simulink model "VoltageSourceConverterHVDCTrans"  (R2025b)
settings: Solver=FixedStepDiscrete  StartTime=0.0  StopTime=5  FixedStep=Ts  MaxStep=1e-4  RelTol=1e-3
PreLoadFcn:
  | VoltageSourceConverterHVDCTransParameters
values from neighbouring files (symbols this model uses):
  c = 0.207e-6    (= 2.07e-07)    [VoltageSourceConverterHVDCTransParameters.m]
  Cf = ((QRatedFilter/(VRated^2*(2*pi*FRated)))*(n^2-1)/(n^2))/Cbase    [VoltageSourceConverterHVDCTransParameters.m]
  FRated = 60    [VoltageSourceConverterHVDCTransParameters.m]
  Idcbase = Pbase/VdcRated    (= 1000)    [VoltageSourceConverterHVDCTransParameters.m]
  IL0 = opIdc.get("I").Value.value    [VoltageSourceConverterHVDCTransInitializeModel.m]
  l = 0.189e-3    (= 0.000189)    [VoltageSourceConverterHVDCTransParameters.m]
  Lbase = Zbase/wbase    [VoltageSourceConverterHVDCTransParameters.m]
  Lr = 0.15    [VoltageSourceConverterHVDCTransParameters.m]
  n = 25    [VoltageSourceConverterHVDCTransParameters.m]
  PRated = 300e6    (= 300000000)    [VoltageSourceConverterHVDCTransParameters.m]
  r = 0.0376    [VoltageSourceConverterHVDCTransParameters.m]
  Rc = r*Dis    (= 11.28)    [VoltageSourceConverterHVDCTransParameters.m]
  Rr = 0.002    [VoltageSourceConverterHVDCTransParameters.m]
  Rt = 0.002625    [VoltageSourceConverterHVDCTransParameters.m]
  Ts = 1/(fsw*100)    [VoltageSourceConverterHVDCTransInitializeModel.m]    (also in VoltageSourceConverterHVDCTransParameters.m = 6.66666666667e-05; VoltageSourceConverterHVDCTransVariantControl.m)
  Tsc = 10*Ts    (= 0.166666666667)    [VoltageSourceConverterHVDCTransInitializeModel.m]    (also in VoltageSourceConverterHVDCTransParameters.m = 6.66666666667e-05; VoltageSourceConverterHVDCTransVariantControl.m)
  Vdcr0 = 2*opReceivingEndVdcp.get("V").Value.value    [VoltageSourceConverterHVDCTransInitializeModel.m]
  VdcRated = 300e3    (= 300000)    [VoltageSourceConverterHVDCTransParameters.m]
  Vdcs0 = 2*opSendingEndVdcp.get("V").Value.value    [VoltageSourceConverterHVDCTransInitializeModel.m]
  VRated = 150e3    (= 150000)    [VoltageSourceConverterHVDCTransParameters.m]
  Xt = 0.19197    [VoltageSourceConverterHVDCTransParameters.m]
  Zbase = Vbase/Ibase    [VoltageSourceConverterHVDCTransParameters.m]
undefined symbols (not defined in the file or in its folder): DiscIntNeverNeededParam
libraries: nesl_utility x43, fl_lib x32, ee_lib x22, eeTransforms x16, eeGeneralControl x14, slpidlib x13, mcbeeMathTransformLib x8, eeSinusoidalMeasurement x2, eePwmGeneratorThreeLevel x2
(part 1 of 4)
CloseFcn:
  | try,close(h1_VoltageSourceConverterHVDCTrans),end
  | clear h1_VoltageSourceConverterHVDCTrans
  | 
  | clear
settings Model: Creator=The MathWorks, Inc.  LastModifiedBy=Elvin
settings DataIOCC: InspectSignalLogs=on  ReturnWorkspaceOutputs=off  SignalLoggingName=logsout_VoltageSourceConverterHVDCTrans
settings DebuggingCC: SubsystemReferenceDiagnosticForUnitTest=warning
settings RTWCC: GPUComputeCapability=3.5
settings SimscapeCC: SimscapeLogType=all  SimscapeLogName=simlog_VoltageSourceConverterHVDCTrans  SimscapeLogLimitData=off  SimscapeOperatingPoint=op

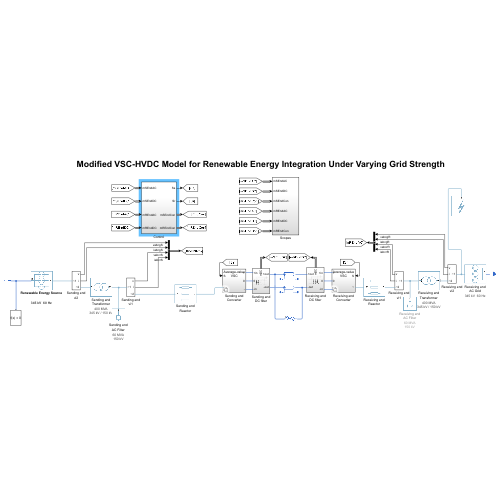
[thumbnail: Simulink's stored preview of the top-level diagram]
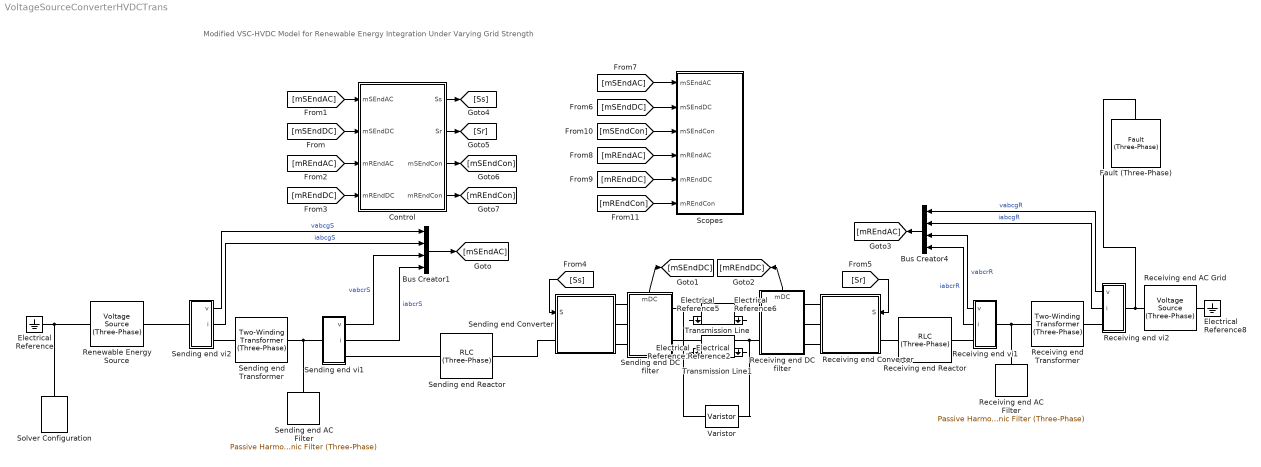
== system VoltageSourceConverterHVDCTrans ==
  note: Modified VSC-HVDC Model for Renewable Energy Integration Under Varying Grid Strength
  Bus Creator1 : BusCreator  Inputs=4
  Bus Creator4 : BusCreator  Inputs=4
  Control : Subsystem
  Electrical Reference{,1..2,5..6,8} (6 alike) : fl_lib/Electrical/Electrical Elements/Electrical Reference
  Fault (Three-Phase) : ee_lib/Utilities/Fault (Three-Phase)  fault_type_option=10  R_pn_fault=0.04 Ohm  R_ng_fault=1e-3 Ohm  exposemeasurement=ee.enum.exposemeasurement.hidden  enable_external_fault=ee.enum.external_fault.hidden  fault_threshold=0.5  fault_condition=1  fault_resettable=0  enable_temporal_fault=1  fault_start_time=2 s  fault_duration=140 ms  G_parasitic=1e-6 1/Ohm
      settings: InternalSimscapePortConfiguration="{\"Bottom\":[],\"Left\":[{\"id\":\"N\",\"label\":\"~\",\"type\":\"foundation.electrical.three_phase\"}],\"Right\":[],\"Top\":[]}"
  Receiving end AC Filter : ee_lib/Passive/Passive Harmonic Filter (Three-Phase)  QRated=QRatedFilter A*V  VRated=VRated V  FRated=FRated Hz  qfactor=15  type_option=ee.enum.filtertype.HPsecondorder  connection_option=ee.enum.filterconnection.Yg  ftuned=n*60 Hz  ftuned1=7 * 60 Hz  ftuned2=11 * 60 Hz  I_specify=off  I_priority=None  I=[0, 0, 0] A  I_nominal_specify=off  I_nominal_value=1  I_nominal_unit=A  V_specify=off  V_priority=None  V=[0, 0, 0] V  V_nominal_specify=off  V_nominal_value=1  V_nominal_unit=V
      settings: InternalSimscapePortConfiguration="{\"Bottom\":[],\"Left\":[{\"id\":\"N\",\"label\":\"~\",\"type\":\"foundation.electrical.three_phase\"}],\"Right\":[],\"Top\":[]}"
      settings: AttributesFormatString=|
      | 60 MVA
      | 150 kV
  Receiving end AC Grid : ee_lib/Sources/Voltage Source (Three-Phase)  vline_rms=VgridRated1 V  shift=0 deg  freq=FRated Hz  impedance_option=1  SShortCircuit=1500e6 A*V  XR=10  R=0.01 Ohm  L=3.97e-4 H  harmonic_option=0  harmonic_orders=[5, 7, 11, 13]  harmonic_ratios=[.1, .1, .1, .1]  G_parasitic=0 1/Ohm  I_specify=on  I_priority=None  I=[0, 0, 0] A  I_nominal_specify=on  I_nominal_value=1  I_nominal_unit=A
      settings: AttributesFormatString="345 kV  60 Hz"
  Receiving end Converter : Subsystem  Variant=on
  Receiving end DC filter : Subsystem
      settings: PortSchema="{\"entries\":[{\"content\":{\"sides\":[{\"content\":{\"connectorIds\":[\"LConn1\",\"LConn2\"]},\"type\":\"ConnectorPlacement.EquallySpacedRectSide\",\"uuid\":\"66d4cfbf-dcba-4749-bf5d-5811a775276e\"},{\"content\":{\"connectorIds\":[\"RConn1\",\"RConn2\",\"RConn3\"],\"side\":\"RIGHT\"},\"type\":\"ConnectorPlacement.EquallySpacedRectSide\",\"uuid\":\"35abdffa-cda0-46f2-9903-3f86a9532248\"},{\"content\":{\"connectorIds\":[\"Out1\"],\"side\":\"TOP\"},\"type\":\"ConnectorPlacement.EquallySpacedRectSide\",\"uuid\":\"3c5502e5-1b76-444d-b26b-a5789383a319\"}]},\"type\":\"ConnectorPlacement.EquallySpacedConnector\",\"uuid\":\"b78b2c4f-7eb3-43f3-aa61-891430661a3a\"}],\"packageUris\":[\"http://schema.mathworks.com/mf0/Connector/R2020b\"],\"version\":\"1.0\"}"
  Receiving end Reactor : ee_lib/Passive/RLC Assemblies/RLC (Three-Phase)  port_option=ee.enum.threePhasePort.composite  component_structure=ee.enum.rlc.structure.SeriesRL  R=Rr*Zbase Ohm  L=Lr*Lbase H  C=1e-6 F  R_parasitic=0 Ohm  G_parasitic=0 1/Ohm  IL_specify=off  IL_priority=High  IL=[0, 0, 0] A  IL_nominal_specify=on  IL_nominal_value=1  IL_nominal_unit=A  VC_specify=off  VC_priority=High  VC=[0, 0, 0] V  VC_nominal_specify=off  VC_nominal_value=1  VC_nominal_unit=V
      settings: InternalSimscapePortConfiguration="{\"Bottom\":[],\"Left\":[{\"id\":\"N1\",\"label\":\"~1\",\"type\":\"foundation.electrical.three_phase\"}],\"Right\":[{\"id\":\"N2\",\"label\":\"~2\",\"type\":\"foundation.electrical.three_phase\"}],\"Top\":[]}"
  Receiving end Transformer : ee_lib/Passive/Transformers/Two-Winding Transformer (Three-Phase)  SRated=Pnom A*V  FRated=FRated Hz  Winding1Connection=ee.enum.windingconnection.Yg  VRated1=Vt1 V  Winding2Connection=ee.enum.windingconnection.delta1  VRated2=Vt2 V  CoreType=ee.enum.coretype.fivelimb  pu_Rw1=Rt/2  pu_Rw2=Rt/2  leakage_reactance_option=ee.enum.transformer_leakage.include  pu_Xl1=Xt/2  pu_Xl2=Xt/2  magnetizing_resistance_option=ee.enum.transformer_magnetizingResistance.include  pu_Rm=500  magnetizing_reactance_option=ee.enum.transformer_magnetizingReactance.include  saturation_option=ee.enum.transformer_saturation.exclude  pu_Xm=500  current_data=[0, .002, 1, 2]  magnetic_flux_data=[0, 1.2, 1.5, 1.51]  pu_X0=0.5  i1_specify=off  i1_priority=None  i1=[0, 0, 0] A  i1_nominal_specify=off  i1_nominal_value=1  i1_nominal_unit=A  i2_specify=off  i2_priority=None  i2=[0, 0, 0] A  i2_nominal_specify=off  i2_nominal_value=1  i2_nominal_unit=A  phi_specify=off  phi_priority=None  phi=[0, 0, 0]  phi_nominal_specify=off  phi_nominal_value=1  phi_nominal_unit=1  power_dissipated_specify=off  power_dissipated_priority=None  power_dissipated=0 W  power_dissipated_nominal_specify=off  power_dissipated_nominal_value=1  power_dissipated_nominal_unit=W
      settings: InternalSimscapePortConfiguration="{\"Bottom\":[],\"Left\":[{\"id\":\"N1\",\"label\":\"~1\",\"type\":\"foundation.electrical.three_phase\"}],\"Right\":[{\"id\":\"N2\",\"label\":\"~2\",\"type\":\"foundation.electrical.three_phase\"}],\"Top\":[]}"
      settings: AttributesFormatString=|
      | 400 MVA
      | 345 kV / 150 kV
  Receiving end vi1 : Subsystem
  Receiving end vi2 : Subsystem
  Renewable Energy Source : ee_lib/Sources/Voltage Source (Three-Phase)  vline_rms=VgridRated V  shift=0 deg  freq=FRated Hz  impedance_option=1  SShortCircuit=5000e6 A*V  XR=15  R=0.01 Ohm  L=3.97e-4 H  harmonic_option=0  harmonic_orders=[5, 7, 11, 13]  harmonic_ratios=[.1, .1, .1, .1]  G_parasitic=0 1/Ohm  I_specify=off  I_priority=None  I=[0, 0, 0] A  I_nominal_specify=off  I_nominal_value=1  I_nominal_unit=A
      settings: AttributesFormatString="345 kV  60 Hz"
  Scopes : Subsystem
  Sending end AC Filter : ee_lib/Passive/Passive Harmonic Filter (Three-Phase)  QRated=QRatedFilter A*V  VRated=VRated V  FRated=FRated Hz  qfactor=15  type_option=ee.enum.filtertype.HPsecondorder  connection_option=ee.enum.filterconnection.Yg  ftuned=n*60 Hz  ftuned1=7 * 60 Hz  ftuned2=11 * 60 Hz  I_specify=off  I_priority=None  I=[0, 0, 0] A  I_nominal_specify=off  I_nominal_value=1  I_nominal_unit=A  V_specify=off  V_priority=None  V=[0, 0, 0] V  V_nominal_specify=off  V_nominal_value=1  V_nominal_unit=V
      settings: InternalSimscapePortConfiguration="{\"Bottom\":[],\"Left\":[{\"id\":\"N\",\"label\":\"~\",\"type\":\"foundation.electrical.three_phase\"}],\"Right\":[],\"Top\":[]}"
      settings: AttributesFormatString=|
      | 60 MVA
      | 150 kV
  Sending end Converter : Subsystem  Variant=on
  Sending end DC filter : Subsystem
      settings: PortSchema="{\"entries\":[{\"content\":{\"sides\":[{\"content\":{\"connectorIds\":[\"LConn1\",\"LConn2\",\"LConn3\"]},\"type\":\"ConnectorPlacement.EquallySpacedRectSide\",\"uuid\":\"66d4cfbf-dcba-4749-bf5d-5811a775276e\"},{\"content\":{\"connectorIds\":[\"RConn1\",\"RConn2\"],\"side\":\"RIGHT\"},\"type\":\"ConnectorPlacement.EquallySpacedRectSide\",\"uuid\":\"35abdffa-cda0-46f2-9903-3f86a9532248\"},{\"content\":{\"connectorIds\":[\"Out1\"],\"side\":\"TOP\"},\"type\":\"ConnectorPlacement.EquallySpacedRectSide\",\"uuid\":\"3c5502e5-1b76-444d-b26b-a5789383a319\"}]},\"type\":\"ConnectorPlacement.EquallySpacedConnector\",\"uuid\":\"b78b2c4f-7eb3-43f3-aa61-891430661a3a\"}],\"packageUris\":[\"http://schema.mathworks.com/mf0/Connector/R2020b\"],\"version\":\"1.0\"}"
  Sending end Reactor : ee_lib/Passive/RLC Assemblies/RLC (Three-Phase)  port_option=ee.enum.threePhasePort.composite  component_structure=ee.enum.rlc.structure.SeriesRL  R=Rr*Zbase Ohm  L=Lr*Lbase H  C=1e-6 F  R_parasitic=0 Ohm  G_parasitic=0 1/Ohm  IL_specify=off  IL_priority=High  IL=[0, 0, 0] A  IL_nominal_specify=on  IL_nominal_value=1  IL_nominal_unit=A  VC_specify=off  VC_priority=High  VC=[0, 0, 0] V  VC_nominal_specify=off  VC_nominal_value=1  VC_nominal_unit=V
      settings: InternalSimscapePortConfiguration="{\"Bottom\":[],\"Left\":[{\"id\":\"N1\",\"label\":\"~1\",\"type\":\"foundation.electrical.three_phase\"}],\"Right\":[{\"id\":\"N2\",\"label\":\"~2\",\"type\":\"foundation.electrical.three_phase\"}],\"Top\":[]}"
  Sending end Transformer : ee_lib/Passive/Transformers/Two-Winding Transformer (Three-Phase)  SRated=Pnom A*V  FRated=FRated Hz  Winding1Connection=ee.enum.windingconnection.Yg  VRated1=Vt1 V  Winding2Connection=ee.enum.windingconnection.delta1  VRated2=Vt2 V  CoreType=ee.enum.coretype.fivelimb  pu_Rw1=Rt/2  pu_Rw2=Rt/2  leakage_reactance_option=ee.enum.transformer_leakage.include  pu_Xl1=Xt/2  pu_Xl2=Xt/2  magnetizing_resistance_option=ee.enum.transformer_magnetizingResistance.include  pu_Rm=500  magnetizing_reactance_option=ee.enum.transformer_magnetizingReactance.include  saturation_option=ee.enum.transformer_saturation.exclude  pu_Xm=500  current_data=[0, .002, 1, 2]  magnetic_flux_data=[0, 1.2, 1.5, 1.51]  pu_X0=0.5  i1_specify=off  i1_priority=None  i1=[0, 0, 0] A  i1_nominal_specify=off  i1_nominal_value=1  i1_nominal_unit=A  i2_specify=off  i2_priority=None  i2=[0, 0, 0] A  i2_nominal_specify=off  i2_nominal_value=1  i2_nominal_unit=A  phi_specify=off  phi_priority=None  phi=[0, 0, 0]  phi_nominal_specify=off  phi_nominal_value=1  phi_nominal_unit=1  power_dissipated_specify=off  power_dissipated_priority=None  power_dissipated=0 W  power_dissipated_nominal_specify=off  power_dissipated_nominal_value=1  power_dissipated_nominal_unit=W
      settings: InternalSimscapePortConfiguration="{\"Bottom\":[],\"Left\":[{\"id\":\"N1\",\"label\":\"~1\",\"type\":\"foundation.electrical.three_phase\"}],\"Right\":[{\"id\":\"N2\",\"label\":\"~2\",\"type\":\"foundation.electrical.three_phase\"}],\"Top\":[]}"
      settings: AttributesFormatString=|
      | 400 MVA
      | 345 kV / 150 kV
  Sending end vi1 : Subsystem
  Sending end vi2 : Subsystem
  Solver Configuration : nesl_utility/Solver Configuration  PhysicalDomain=network_engine_domain  SubClassName=solver  LeftPortType=input  RightPortType=generic  Tones=[]  Harmonics=[]  SimulateNoise=off  Profile=off  UseLocalSampling=off  EnableSwitchedLinearOptims=on  FrequencyDomain=off  UseCCode=off  RelTol=0.001  AbsTol=0.001  MinStep=1e-09  ToWorkspace=off  RevertToSquareIcSolve=off  NumHomotopyIterations=100  PhasorMode=off  PhasorModeNumHarmonics=1  ConsistencySolver=NEWTON_XTOL_AFTER_FTOL  IndexReductionMethod=DerivativeReplacement  DoDC=on  ResidualTolerance=1e-09  ConsistencyTolSource=GLOBAL  ConsistencyAbsTol=0.001  ConsistencyRelTol=0.001  ConsistencyTolFactor=0.001  UseLocalSolver=on  LocalSolverChoice=NE_BACKWARD_EULER_ADVANCER  ResolveIndetEquations=on  FunctionEvalNumThread=1  LocalSolverSampleTime=Ts  DoFixedCost=on  MaxNonlinIter=3  MaxModeIter=2  ComputeImpulses=off  ImpulseIterations=2  LinearAlgebra=auto  LinearAlgebraNumThread=0  EquationFormulation=NE_TIME_EF  DelaysMemoryBudget=1024  AutomaticFiltering=on  FilteringTimeConstant=0.001  PartitionStorageMethod=AS_NEEDED  PartitionMemoryBudget=1024  PartitionMethod=ROBUST  MultibodyUseLocalSolver=off  MultibodyLocalSolverChoice=ODE1  MultibodyLocalSolverSampleTime=0.001
  Transmission Line : ee_lib/Passive/Lines/Transmission Line  model_type=4  TD=5 ns  LC_param=2  Z0_delay_based=50 Ohm  Z0=50 Ohm  freq=FRated Hz  Ll=l*1e-3 H/m  L=l H/km  C=c F/km  R=r Ohm/km  G=0 S/km  LEN=Dis km  N=1
      settings: InternalSimscapePortConfiguration="{\"Bottom\":[],\"Left\":[{\"id\":\"p1\",\"label\":\"\",\"type\":\"foundation.electrical.electrical\"},{\"id\":\"n1\",\"label\":\"\",\"type\":\"foundation.electrical.electrical\"}],\"Right\":[{\"id\":\"p2\",\"label\":\"\",\"type\":\"foundation.electrical.electrical\"},{\"id\":\"n2\",\"label\":\"\",\"type\":\"foundation.electrical.electrical\"}],\"Top\":[]}"
  Transmission Line1 : ee_lib/Passive/Lines/Transmission Line  model_type=4  TD=5 ns  LC_param=2  Z0_delay_based=50 Ohm  Z0=50 Ohm  freq=FRated Hz  Ll=l*1e-3 H/m  L=l H/km  C=c F/km  R=r Ohm/km  G=0 S/km  LEN=Dis km  N=1
      settings: InternalSimscapePortConfiguration="{\"Bottom\":[],\"Left\":[{\"id\":\"p1\",\"label\":\"\",\"type\":\"foundation.electrical.electrical\"},{\"id\":\"n1\",\"label\":\"\",\"type\":\"foundation.electrical.electrical\"}],\"Right\":[{\"id\":\"p2\",\"label\":\"\",\"type\":\"foundation.electrical.electrical\"},{\"id\":\"n2\",\"label\":\"\",\"type\":\"foundation.electrical.electrical\"}],\"Top\":[]}"
  Varistor : ee_lib/Passive/Varistor  prm=ee.enum.passive.varistor.varistorParameterization.powerLaw  vclamp=260 V  roff=3e8 Ohm  ron=1 Ohm  vln=330e3 V  vnu=450e3 V  rLeak=3e8 Ohm  alphaNormal=30  rUpturn=5 Ohm  rseries=100e-6 Ohm  c=0 nF  v_varistor_specify=off  v_varistor_priority=None  v_varistor=0 V  v_varistor_nominal_specify=off  v_varistor_nominal_value=1  v_varistor_nominal_unit=V
      settings: InternalSimscapePortConfiguration="{\"Bottom\":[],\"Left\":[{\"id\":\"p\",\"label\":\"+\",\"type\":\"foundation.electrical.electrical\"}],\"Right\":[{\"id\":\"n\",\"label\":\"-\",\"type\":\"foundation.electrical.electrical\"}],\"Top\":[]}"
  wires:
  Sending end vi2/1(v) -> Bus Creator1/1  "vabcgS"
  Sending end vi2/2(i) -> Bus Creator1/2  "iabcgS"
  Bus Creator1/1 -> [mSEndAC]
  [mSEndAC] -> Control/1(mSEndAC)
  Sending end vi1/1(v) -> Bus Creator1/3  "vabcrS"
  Sending end vi1/2(i) -> Bus Creator1/4  "iabcrS"
  [mSEndDC] -> Control/2(mSEndDC)
  Receiving end DC filter/1(mDC) -> [mREndDC]
  Receiving end vi2/1(v) -> Bus Creator4/1  "vabcgR"
  Receiving end vi2/2(i) -> Bus Creator4/2  "iabcgR"
  Receiving end vi1/1(v) -> Bus Creator4/3  "vabcrR"
  Receiving end vi1/2(i) -> Bus Creator4/4  "iabcrR"
  Bus Creator4/1 -> [mREndAC]
  [mREndAC] -> Control/3(mREndAC)
  [mREndDC] -> Control/4(mREndDC)
  Control/1(Ss) -> [Ss]
  Control/2(Sr) -> [Sr]
  [Ss] -> Sending end Converter/1(S)
  [Sr] -> Receiving end Converter/1(S)
  Control/3(mSEndCon) -> [mSEndCon]
  Control/4(mREndCon) -> [mREndCon]
  [mSEndAC] -> Scopes/1(mSEndAC)
  [mSEndDC] -> Scopes/2(mSEndDC)
  [mSEndCon] -> Scopes/3(mSEndCon)
  [mREndAC] -> Scopes/4(mREndAC)
  [mREndDC] -> Scopes/5(mREndDC)
  [mREndCon] -> Scopes/6(mREndCon)
  Sending end DC filter/1(mDC) -> [mSEndDC]
  connections:
  Renewable Energy Source/RConn1 -- Sending end vi2/LConn1
  Sending end Transformer/LConn1 -- Sending end vi2/RConn1
  Sending end Converter/LConn1 -- Sending end Reactor/RConn1
  Sending end AC Filter/LConn1 -- Sending end Transformer/RConn1 -- Sending end vi1/LConn1
  Sending end vi1/RConn1 -- Sending end Reactor/LConn1
  Sending end DC filter/LConn2 -- Sending end Converter/RConn2
  Receiving end Converter/LConn1 -- Receiving end Reactor/RConn1
  Receiving end vi1/RConn1 -- Receiving end Reactor/LConn1
  Receiving end AC Filter/LConn1 -- Receiving end Transformer/RConn1 -- Receiving end vi1/LConn1
  Receiving end Transformer/LConn1 -- Receiving end vi2/RConn1
  Receiving end AC Grid/LConn1 -- Electrical Reference8/LConn1
  Receiving end AC Grid/RConn1 -- Fault (Three-Phase)/LConn1 -- Receiving end vi2/LConn1
  Transmission Line/LConn1 -- Varistor/LConn1 -- Sending end DC filter/RConn1
  Transmission Line1/LConn1 -- Sending end DC filter/RConn2
  Electrical Reference/LConn1 -- Renewable Energy Source/LConn1 -- Solver Configuration/RConn1
  Transmission Line/RConn2 -- Electrical Reference6/LConn1
  Transmission Line/LConn2 -- Electrical Reference5/LConn1
  Sending end DC filter/LConn3 -- Sending end Converter/RConn3
  Sending end DC filter/LConn1 -- Sending end Converter/RConn1
  Transmission Line1/RConn1 -- Varistor/RConn1 -- Receiving end DC filter/LConn2
  Receiving end DC filter/RConn1 -- Receiving end Converter/RConn1
  Receiving end DC filter/RConn2 -- Receiving end Converter/RConn2
  Receiving end DC filter/RConn3 -- Receiving end Converter/RConn3
  Transmission Line/RConn1 -- Receiving end DC filter/LConn1
  Transmission Line1/RConn2 -- Electrical Reference2/LConn1
  Transmission Line1/LConn2 -- Electrical Reference1/LConn1

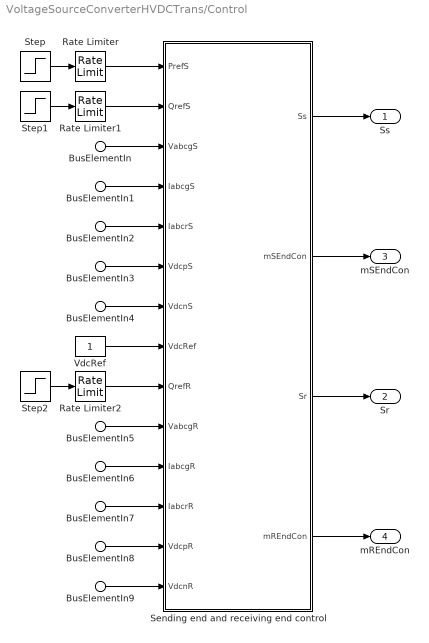
== system VoltageSourceConverterHVDCTrans/Control ==
  BusElementIn : Inport  PortName=mSEndAC  Element=vabcgS
  BusElementIn1 : Inport  PortName=mSEndAC  Element=iabcgS
  BusElementIn2 : Inport  PortName=mSEndAC  Element=iabcrS
  BusElementIn3 : Inport  Port=2  PortName=mSEndDC  Element=VdcpS
  BusElementIn4 : Inport  Port=2  PortName=mSEndDC  Element=VdcnS
  BusElementIn5 : Inport  Port=3  PortName=mREndAC  Element=vabcgR
  BusElementIn6 : Inport  Port=3  PortName=mREndAC  Element=iabcgR
  BusElementIn7 : Inport  Port=3  PortName=mREndAC  Element=iabcrR
  BusElementIn8 : Inport  Port=4  PortName=mREndDC  Element=VdcpR
  BusElementIn9 : Inport  Port=4  PortName=mREndDC  Element=VdcnR
  Rate Limiter : RateLimiter  RisingSlewLimit=1.0  FallingSlewLimit=0  SampleTimeMode=inherited  InitialCondition=1.0
  Rate Limiter1 : RateLimiter  RisingSlewLimit=0.2  FallingSlewLimit=0  SampleTimeMode=inherited  InitialCondition=0.2
  Rate Limiter2 : RateLimiter  RisingSlewLimit=0  FallingSlewLimit=-0.2  SampleTimeMode=inherited  InitialCondition=-0.2
  Sending end and receiving end control : Subsystem  mask{PRated=PRated, VRated=VRated, FRated=FRated, VdcRated=VdcRated, TranRL=[Rt Xt], Cf=Cf, ReRL=[Rr Lr], Rc=Rc, Ts=Ts, Tsc=Tsc, modeling_fidelity=Medium, InitUsingOP=off, SEnd_Pref=1.0, SEnd_Qref=0.2, SEnd_P_PI_Low=[0.19  22.74], SEnd_Q_PI_Low=[0.76  35.86], SEnd_P_PI=[0 29.14], SEnd_Q_PI=[0 29.51], SEnd_Id_PI=[0.5035  3.648], SEnd_Iq_PI=[0.4291  5.154], Vabcgs0=[-0.030405    -0.85315     0.88355], Vphases0=-0.030315, Vdqgs0=[1.0031           0], Iabcgs0=[0.084538    -0.47634      0.3918], Idqgs0=[0.49843    0.099691], Iabcrs0=[-0.33786    -0.13774      0.4756], Idqs0=[0.47888    -0.10107], P_PIs0=0.49843, Q_PIs0=0.099691, Id_PIs0=0.0046314, Iq_PIs0=3.8914e-05, Vdcs0=303702.7829, IL0=492.3913, REnd_VdcRef=1, REnd_Qref=-0.2, REnd_Vdc_PI_Low=[1.52  9.15], REnd_Q_PI_Low=[0.74  35.13], REnd_Vdc_PI=[0.71  11.03], REnd_Q_PI=[0.0013  39.17], REnd_Id_PI=[0.65  4.59], REnd_Iq_PI=[0.90  6.33], REnd_VdcB_P=2, Vabcgr0=[0.028242    -0.88656     0.85832], Vphaser0=0.028027, Vdqgr0=[1.0078           0], Iabcgr0=[0.085848     0.37156    -0.45741], Idqgr0=[-0.47601    0.099226], Iabcrr0=[0.13027     0.33314    -0.46341], Idqr0=[-0.46651     -0.1041], P_PIr0=-0.47601, Q_PIr0=0.099226, Id_PIr0=-0.0047674, Iq_PIr0=4.0379e-05, Vdcr0=300000}
      mask prompts: PRated "Rated power (W)"; VRated "Rated AC voltage, rms line-to-line (V)"; FRated "Grid frequency (Hz)"; VdcRated "Rated DC voltage (V)"; TranRL "Transformer winding resistance and leakage inductance (pu)"; Cf "AC filter capacitance (pu)"; ReRL "Reactor resistance and inductance (pu)"; Rc "Transmission line total resistance (Ohm)"; Ts "Fundamental sample time (s)"; Tsc "Control sample time (s)"; modeling_fidelity "Modeling fidelity level"; InitUsingOP "Initialize control using Simscape operating point"; SEnd_Pref "Active power reference (pu)"; SEnd_Qref "Reactive power reference (pu)"; SEnd_P_PI_Low "Active power control proportional and integral gain"; SEnd_Q_PI_Low "Reactive power control proportional and integral gain"; SEnd_P_PI "Active power control proportional and integral gain"; SEnd_Q_PI "Reactive power control proportional and integral gain"; SEnd_Id_PI "D-axis current control proportional and integral gain"; SEnd_Iq_PI "Q-axis current control proportional and integral gain"; Vabcgs0 "Initial three-phase AC grid voltage (pu)"; Vphases0 "Initial phase angle of Phase-A voltage (rad)"; Vdqgs0 "Initial dq-axes grid voltage (pu)"; Iabcgs0 "Initial three-phase AC grid current (pu)"; Idqgs0 "Initial dq-axes grid current (pu)"; Iabcrs0 "Initial three-phase reactor current (pu)"; Idqs0 "Initial dq-axes reactor current (pu)"; P_PIs0 "Initial state of active power PI (pu)"; Q_PIs0 "Initial state of reactive power PI (pu)"; Id_PIs0 "Initial state of d-axis current PI (pu)"; Iq_PIs0 "Initial state of q-axis current PI (pu)"; Vdcs0 "Initial sending-end DC voltage (V)"; IL0 "Initial DC current (A)"; REnd_VdcRef "DC voltage reference (pu)"; REnd_Qref "Reactive power reference (pu)"; REnd_Vdc_PI_Low "DC voltage control proportional and integral gain"; REnd_Q_PI_Low "Reactive power control proportional and integral gain"; REnd_Vdc_PI "DC voltage control proportional and integral gain"; REnd_Q_PI "Reactive power control proportional and integral gain"; REnd_Id_PI "D-axis current control proportional and integral gain"; REnd_Iq_PI "Q-axis current control proportional and integral gain"; REnd_VdcB_P "DC voltage balancing control proportional gain"; Vabcgr0 "Initial three-phase AC grid voltage (pu)"; Vphaser0 "Initial phase angle of Phase-A voltage (rad)"; Vdqgr0 "Initial dq-axes grid voltage (pu)"; Iabcgr0 "Initial three-phase AC grid current (pu)"; Idqgr0 "Initial dq-axes grid current (pu)"; Iabcrr0 "Initial three-phase reactor current (pu)"; Idqr0 "Initial dq-axes reactor current (pu)"; P_PIr0 "Initial state of DC voltage PI (pu)"; Q_PIr0 "Initial state of reactive power PI (pu)"; Id_PIr0 "Initial state of d-axis current PI (pu)"; Iq_PIr0 "Initial state of q-axis current PI (pu)"; Vdcr0 "Initial receiving-end DC voltage (V)"
      mask init:
      | Pbase = PRated; % base power
      | Vbase = VRated/sqrt(3)*sqrt(2); % base voltage
      | wbase = 2*pi*FRated; % base elec. radial frequency
      | 
      | Rt = TranRL(1); % pu, transformer total resistance
      | Lt = TranRL(2); % pu, transformer total leakage inductance
      | Rr = ReRL(1); % pu, reactor resistance
      | Lr = ReRL(2); % pu, reactor inductance
      | 
      | if strcmp(get_param(gcb,'InitUsingOP'),'off')
      |     % Sending end
      |     Ps0 = SEnd_Pref; % pu, sending end grid active power
      |     Qs0 = SEnd_Qref; % pu, sending end grid reactive power
      |     Vphases0 = 0; % rad, initial phase angle of Phase-A voltage
      |     Vdgs0 = 1; % pu, d-axis grid voltage
      |     Vqgs0 = 0; % pu, q-axis grid voltage
      |     Vabcgs0 = Vdgs0*sin(Vphases0+[0 -1 1]*2*pi/3); % pu, initial three-phase AC grid voltage
      |     Idgs0 = Ps0/Vdgs0; % pu, d-axis grid current
      |     Iqgs0 = -Qs0/Vdgs0; % pu, q-axis grid current
      |     Iabcgs0 = ([sin(Vphases0) cos(Vphases0);...
      |         sin(Vphases0-2*pi/3) cos(Vphases0-2*pi/3);...
      |         sin(Vphases0+2*pi/3) cos(Vphases0+2*pi/3)] * [Idgs0;Iqgs0])'; % pu, initial three-phase AC grid current
      |     Vdfs0 = Vdgs0 - Rt*Idgs0 + Lt*Iqgs0; % pu, d-axis filter terminal voltage
      |     Vqfs0 = Vqgs0 - Rt*Iqgs0 - Lt*Idgs0; % pu, q-axis filter terminal voltage
      |     Ids0 = Idgs0 + Cf*Vqfs0; % pu, d-axis reactor current
      |     Iqs0 = Iqgs0 - Cf*Vdfs0; % pu, q-axis reactor current
      |     Iabcrs0 = ([sin(-pi/6+Vphases0) cos(-pi/6+Vphases0);...
      |         sin(-pi/6+Vphases0-2*pi/3) cos(-pi/6+Vphases0-2*pi/3);...
      |         sin(-pi/6+Vphases0+2*pi/3) cos(-pi/6+Vphases0+2*pi/3)] * [Ids0;Iqs0])'; % pu, initial three-phase reactor current
      |     Vds0 = Vdfs0 - Rr*Ids0 + Lr*Iqs0; % pu, d-axis converter voltage
      |     Vqs0 = Vqfs0 - Rr*Iqs0 - Lr*Ids0; % pu, q-axis converter voltage
      |     Pcs0 = Vqs0*Iqs0 + Vds0*Ids0; % pu, sending end active power flowing into the converter
      |     Id_PIs0 = (Vdgs0+Iqgs0*Lt+Iqs0*Lr) - Vds0; % pu, d-axis current PI initial state
      |     Iq_PIs0 = -(Idgs0*Lt+Ids0*Lr) - Vqs0; % pu, q-axis current PI initial state
      |     P_PIs0 = Idgs0; % pu, active power PI initial state
      |     Q_PIs0 = Iqgs0; % pu, reactive power PI initial state
      | 
      |     % DC side
      |     Vdcr0 = VdcRated*REnd_VdcRef; % V, receiving end DC voltage
      |     Vdcs0 = 0.5*(Vdcr0+sqrt(Vdcr0^2+4*Pcs0*Pbase*(2*Rc))); % V, sending end DC voltage
      |     IL0 = Pcs0*Pbase/Vdcs0; % A, DC current
      |     Pcr0 = -Vdcr0*IL0/Pbase; % pu, receiving end active power flowing into the converter
      | 
      |     % Receiving end
      |     Qr0 = REnd_Qref; % pu, receiving end grid reactive power
      |     Vphaser0 = 0; % rad, initial phase angle of Phase-A voltage
      |     Vdgr0 = 1; % pu, d-axis grid voltage
      |     Vqgr0 = 0; % pu, q-axis grid voltage
      |     Vabcgr0 = Vdgr0*sin(Vphaser0+[0 -1 1]*2*pi/3); % pu, initial three-phase AC grid voltage
      |     Iqgr0 = -Qr0/Vdgr0; % pu, q-axis grid current
      | 
      |     coefA = ((-Lt*(1-Lr*Cf)-Rr*Cf*Rt-Lr)*Rt*Cf + (-Rt*(1-Lr*Cf)+Rr*Cf*Lt-Rr)*(1-Cf*Lt));
      |     coefB = (Rr*Cf^2*Rt+(-Lt*(1-Lr*Cf)-Rr*Cf*Rt-Lr)*(-Cf)+(1-Lr*Cf)*(1-Cf*Lt))*Vdgr0;
      |     coefC = -Rr*Cf^2*Vdgr0^2 + ...
      |         ((-Rt*(1-Lr*Cf)+Rr*Cf*Lt-Rr)*(1-Cf*Lt)+(Lt*(1-Lr*Cf)+Rr*Cf*Rt+Lr)*(-Rt*Cf))*Iqgr0^2 + ...
      |         (Rr*Cf*(1-Cf*Lt)+(-Rt*(1-Lr*Cf)+Rr*Cf*Lt-Rr)*(-Cf)+(1-Lr*Cf)*(-Rt*Cf))*Vdgr0*Iqgr0 - Pcr0;
      |     Idgr0 = (-coefB+sqrt(coefB^2-4*coefA*coefC))/2/coefA; % pu, d-axis grid current
      |     Iabcgr0 = ([sin(Vphaser0) cos(Vphaser0);...
      |         sin(Vphaser0-2*pi/3) cos(Vphaser0-2*pi/3);...
      |         sin(Vphaser0+2*pi/3) cos(Vphaser0+2*pi/3)] * [Idgr0;Iqgr0])'; % pu, initial three-phase AC current
      |     Pr0 = Idgr0*Vdgr0;
      |     Vdfr0 = Vdgr0 - Rt*Idgr0 + Lt*Iqgr0; % pu, d-axis filter terminal voltage
      |     Vqfr0 = Vqgr0 - Rt*Iqgr0 - Lt*Idgr0; % pu, q-axis filter terminal voltage
      |     Idr0 = Idgr0 + Cf*Vqfr0; % pu, d-axis reactor current
      |     Iqr0 = Iqgr0 - Cf*Vdfr0; % pu, q-axis reactor current
      |     Iabcrr0 = ([sin(-pi/6+Vphaser0) cos(-pi/6+Vphaser0);...
      |         sin(-pi/6+Vphaser0-2*pi/3) cos(-pi/6+Vphaser0-2*pi/3);...
      |         sin(-pi/6+Vphaser0+2*pi/3) cos(-pi/6+Vphaser0+2*pi/3)]*[Idr0;Iqr0])'; % pu
      |     Vdr0 = Vdfr0 - Rr*Idr0 + Lr*Iqr0; % pu, d-axis converter voltage
      |     Vqr0 = Vqfr0 - Rr*Iqr0 - Lr*Idr0; % pu, q-axis converter voltage
      |     Id_PIr0 = (Vdgr0+Iqgr0*Lt+Iqr0*Lr) - Vdr0; % pu, d-axis current PI initial state
      |     Iq_PIr0 = -(Idgr0*Lt+Idr0*Lr) - Vqr0; % pu, q-axis current PI initial state
      |     P_PIr0 = Idgr0; % pu, active power PI initial state
      |     Q_PIr0 = Iqgr0; % pu, reactive power PI initial state
      | 
      |     assignin('base','IL0',IL0);
      |     assignin('base','Vdcr0',Vdcr0);
      |     assignin('base','Vdcs0',Vdcs0);
      | 
      | else
      | 
      |  if strcmp(get_param(bdroot,'SimscapeUseOperatingPoints'),'on')
      |    Vdgs0 = Vdqgs0(1);
      |    Vqgs0 = Vdqgs0(2);
      |    Idgs0 = Idqgs0(1);
      |    Iqgs0 = Idqgs0(2);   
      |    Ids0 = Idqs0(1);
      |    Iqs0 = Idqs0(2); 
      | 
      |    Vdgr0 = Vdqgr0(1);
      |    Vqgr0 = Vdqgr0(2);
      |    Idgr0 = Idqgr0(1);
      |    Iqgr0 = Idqgr0(2);   
      |    Idr0 = Idqr0(1);
      |    Iqr0 = Idqr0(2); 
      | 
      |    Ps0 = SEnd_Pref;
      |    Qs0 = SEnd_Qref;
      |    Qr0 = REnd_Qref;
      |  else
      |    warning('Please execute ''Initialize model using Simscape operating point''') 
      |  end
      | 
      | end
      mask TypeOptions modeling_fidelity: Low | Medium | High
      mask Callback modeling_fidelity:
      | switch get_param(gcb,'modeling_fidelity')
      |     case 'Low'
      |         set_param(gcb,'MaskVisibilities',{'on';'on';'on';'on';'on';'on';'on';'on';'on';'on';'on';'on';...
      |             'on';'on';'on';'on';'off';'off';'off';'off';...
      |             'off';'off';'off';'off';'off';'off';'off';'off';'off';'off';'off';'off';'off';...
      |             'on';'on';'on';'on';'off';'off';'off';'off';'off';...
      |             'off';'off';'off';'off';'off';'off';'off';'off';'off';'off';'off';'off'})
      |     case 'Medium'
      |         set_param(gcb,'MaskVisibilities',{'on';'on';'on';'on';'on';'on';'on';'on';'on';'on';'on';'on';...
      |             'on';'on';'off';'off';'on';'on';'on';'on';...
      |             'off';'off';'off';'off';'off';'off';'off';'off';'off';'off';'off';'off';'off';...
      |             'on';'on';'off';'off';'on';'on';'on';'on';'off';...
      |             'off';'off';'off';'off';'off';'off';'off';'off';'off';'off';'off';'off'})
      |     otherwise
      |         set_param(gcb,'MaskVisibilities',{'on';'on';'on';'on';'on';'on';'on';'on';'on';'on';'on';'on';...
      |             'on';'on';'off';'off';'on';'on';'on';'on';...
      |             'off';'off';'off';'off';'off';'off';'off';'off';'off';'off';'off';'off';'off';...
      |             'on';'on';'off';'off';'on';'on';'on';'on';'on';...
      |             'off';'off';'off';'off';'off';'off';'off';'off';'off';'off';'off';'off'})
      | end
      mask DialogControl Container4 Prompt: System
      mask DialogControl Container5 Prompt: Sending End Control
      mask DialogControl Container6 Prompt: Receiving End Control
  Step : Step  Time=0  Before=1.0  After=1.0  SampleTime=0
  Step1 : Step  Time=0  Before=0.2  After=0.2  SampleTime=0
  Step2 : Step  Time=0  Before=-0.2  After=-0.2  SampleTime=0
  VdcRef : Constant  SampleTime=0
  Ss : Outport
  Sr : Outport  Port=2
  mSEndCon : Outport  Port=3
  mREndCon : Outport  Port=4
  wires:
  Step/1 -> Rate Limiter/1
  Step1/1 -> Rate Limiter1/1
  Step2/1 -> Rate Limiter2/1
  Rate Limiter/1 -> Sending end and receiving end control/1(PrefS)
  Rate Limiter1/1 -> Sending end and receiving end control/2(QrefS)
  BusElementIn/1 -> Sending end and receiving end control/3(VabcgS)
  BusElementIn1/1 -> Sending end and receiving end control/4(IabcgS)
  BusElementIn2/1 -> Sending end and receiving end control/5(IabcrS)
  BusElementIn3/1 -> Sending end and receiving end control/6(VdcpS)
  BusElementIn4/1 -> Sending end and receiving end control/7(VdcnS)
  VdcRef/1 -> Sending end and receiving end control/8(VdcRef)
  Rate Limiter2/1 -> Sending end and receiving end control/9(QrefR)
  BusElementIn5/1 -> Sending end and receiving end control/10(VabcgR)
  BusElementIn6/1 -> Sending end and receiving end control/11(IabcgR)
  BusElementIn7/1 -> Sending end and receiving end control/12(IabcrR)
  BusElementIn8/1 -> Sending end and receiving end control/13(VdcpR)
  BusElementIn9/1 -> Sending end and receiving end control/14(VdcnR)
  Sending end and receiving end control/1(Ss) -> Ss/1
  Sending end and receiving end control/2(mSEndCon) -> mSEndCon/1
  Sending end and receiving end control/3(Sr) -> Sr/1
  Sending end and receiving end control/4(mREndCon) -> mREndCon/1

== system VoltageSourceConverterHVDCTrans/Receiving end Converter ==
  S : Inport
  Average-value VSC : Subsystem  VariantControl=AverageValueVSC
  Switching VSC : Subsystem  VariantControl=SwitchingVSC
  + : PMIOPort  Side=Right
  0 : PMIOPort  Port=2  Side=Right
  - : PMIOPort  Port=3  Side=Right
  ~ : PMIOPort  Port=4  Side=Left

== system VoltageSourceConverterHVDCTrans/Receiving end DC filter ==
  Bus Creator : BusCreator  Inputs=4
  Cfnr : fl_lib/Electrical/Electrical Elements/Capacitor  c=Cdcf F  r=0 Ohm  g=0 1/Ohm  i_specify=off  i_priority=High  i=0 A  i_nominal_specify=off  i_nominal_value=1  i_nominal_unit=A  v_specify=off  v_priority=High  v=Vdcs0/2 V  v_nominal_specify=off  v_nominal_value=1  v_nominal_unit=V  vc_specify=on  vc_priority=High  vc=Vdcr0/2 V  vc_nominal_specify=off  vc_nominal_value=1  vc_nominal_unit=V
  Cfpr : fl_lib/Electrical/Electrical Elements/Capacitor  c=Cdcf F  r=0 Ohm  g=0 1/Ohm  i_specify=off  i_priority=High  i=0 A  i_nominal_specify=off  i_nominal_value=1  i_nominal_unit=A  v_specify=off  v_priority=High  v=Vdcs0/2 V  v_nominal_specify=off  v_nominal_value=1  v_nominal_unit=V  vc_specify=on  vc_priority=High  vc=Vdcr0/2 V  vc_nominal_specify=off  vc_nominal_value=1  vc_nominal_unit=V
  Cnr : fl_lib/Electrical/Electrical Elements/Capacitor  c=Cdc F  r=1e-3 Ohm  g=0 1/Ohm  i_specify=off  i_priority=High  i=0 A  i_nominal_specify=off  i_nominal_value=1  i_nominal_unit=A  v_specify=off  v_priority=High  v=Vdcs0/2 V  v_nominal_specify=off  v_nominal_value=1  v_nominal_unit=V  vc_specify=on  vc_priority=High  vc=Vdcr0/2 V  vc_nominal_specify=off  vc_nominal_value=1  vc_nominal_unit=V
  Cpr : fl_lib/Electrical/Electrical Elements/Capacitor  c=Cdc F  r=1e-3 Ohm  g=0 1/Ohm  i_specify=off  i_priority=High  i=0 A  i_nominal_specify=off  i_nominal_value=1  i_nominal_unit=A  v_specify=off  v_priority=High  v=Vdcs0/2 V  v_nominal_specify=off  v_nominal_value=1  v_nominal_unit=V  vc_specify=on  vc_priority=High  vc=Vdcr0/2 V  vc_nominal_specify=off  vc_nominal_value=1  vc_nominal_unit=V
  Electrical Reference : fl_lib/Electrical/Electrical Elements/Electrical Reference
  Lfnr : fl_lib/Electrical/Electrical Elements/Inductor  l=L2 H  r=0.05 Ohm  g=0 1/Ohm  i_specify=off  i_priority=None  i=0 A  i_nominal_specify=off  i_nominal_value=1  i_nominal_unit=A  v_specify=off  v_priority=None  v=0 V  v_nominal_specify=off  v_nominal_value=1  v_nominal_unit=V  i_L_specify=on  i_L_priority=High  i_L=IL0 A  i_L_nominal_specify=off  i_L_nominal_value=1  i_L_nominal_unit=A
  Lfpr : fl_lib/Electrical/Electrical Elements/Inductor  l=L2 H  r=0.05 Ohm  g=0 1/Ohm  i_specify=off  i_priority=None  i=0 A  i_nominal_specify=off  i_nominal_value=1  i_nominal_unit=A  v_specify=off  v_priority=None  v=0 V  v_nominal_specify=off  v_nominal_value=1  v_nominal_unit=V  i_L_specify=on  i_L_priority=High  i_L=-IL0 A  i_L_nominal_specify=off  i_L_nominal_value=1  i_L_nominal_unit=A
  Lfr : fl_lib/Electrical/Electrical Elements/Inductor  l=L1 H  r=0.1 Ohm  g=0 1/Ohm  i_specify=off  i_priority=None  i=0 A  i_nominal_specify=off  i_nominal_value=1  i_nominal_unit=A  v_specify=off  v_priority=None  v=0 V  v_nominal_specify=off  v_nominal_value=1  v_nominal_unit=V  i_L_specify=on  i_L_priority=None  i_L=0 A  i_L_nominal_specify=off  i_L_nominal_value=1  i_L_nominal_unit=A
  Sensing current1 : Subsystem
      settings: PortSchema="{\"entries\":[{\"content\":{\"sides\":[{\"content\":{\"connectorIds\":[\"LConn1\"]},\"type\":\"ConnectorPlacement.EquallySpacedRectSide\",\"uuid\":\"b182dbc5-c8d5-4832-a7cd-ea3787954646\"},{\"content\":{\"connectorIds\":[\"RConn1\",\"Out1\"],\"side\":\"RIGHT\"},\"type\":\"ConnectorPlacement.EquallySpacedRectSide\",\"uuid\":\"bfc6f163-1abf-440b-aa89-1443f971fd07\"},{\"content\":{\"connectorIds\":[],\"side\":\"TOP\"},\"type\":\"ConnectorPlacement.EquallySpacedRectSide\",\"uuid\":\"dd2a104c-9a72-483e-91c4-dbef9b359450\"}]},\"type\":\"ConnectorPlacement.EquallySpacedConnector\",\"uuid\":\"ce98cc3b-f524-409d-a465-fff2e3b7df79\"}],\"packageUris\":[\"http://schema.mathworks.com/mf0/Connector/R2020b\"],\"version\":\"1.0\"}"
  Sensing current2 : Subsystem
      settings: PortSchema="{\"entries\":[{\"content\":{\"sides\":[{\"content\":{\"connectorIds\":[\"LConn1\"]},\"type\":\"ConnectorPlacement.EquallySpacedRectSide\",\"uuid\":\"b182dbc5-c8d5-4832-a7cd-ea3787954646\"},{\"content\":{\"connectorIds\":[\"RConn1\",\"Out1\"],\"side\":\"RIGHT\"},\"type\":\"ConnectorPlacement.EquallySpacedRectSide\",\"uuid\":\"bfc6f163-1abf-440b-aa89-1443f971fd07\"},{\"content\":{\"connectorIds\":[],\"side\":\"TOP\"},\"type\":\"ConnectorPlacement.EquallySpacedRectSide\",\"uuid\":\"dd2a104c-9a72-483e-91c4-dbef9b359450\"}]},\"type\":\"ConnectorPlacement.EquallySpacedConnector\",\"uuid\":\"ce98cc3b-f524-409d-a465-fff2e3b7df79\"}],\"packageUris\":[\"http://schema.mathworks.com/mf0/Connector/R2020b\"],\"version\":\"1.0\"}"
  Vdcn : Subsystem
      settings: PortSchema="{\"entries\":[{\"content\":{\"sides\":[{\"content\":{\"connectorIds\":[\"LConn1\",\"Out1\"]},\"type\":\"ConnectorPlacement.EquallySpacedRectSide\",\"uuid\":\"bc3757cc-4537-444e-89af-7b7d8c8c1fa7\"},{\"content\":{\"connectorIds\":[\"RConn1\"],\"side\":\"RIGHT\"},\"type\":\"ConnectorPlacement.EquallySpacedRectSide\",\"uuid\":\"908bf4c4-26f6-4d8a-bcf8-68236027f5f8\"},{\"content\":{\"side\":\"TOP\"},\"type\":\"ConnectorPlacement.EquallySpacedRectSide\",\"uuid\":\"33f228db-ba47-4718-96dc-a72de309ae8c\"},{\"content\":{\"side\":\"BOTTOM\"},\"type\":\"ConnectorPlacement.EquallySpacedRectSide\",\"uuid\":\"d9b66c7e-0954-4c47-8bcc-77bf13ff573c\"}]},\"type\":\"ConnectorPlacement.EquallySpacedConnector\",\"uuid\":\"345f3578-0572-4e64-b2f3-84728129a12d\"}],\"packageUris\":[\"http://schema.mathworks.com/mf0/Connector/R2020b\"],\"version\":\"1.0\"}"
  Vdcp : Subsystem
      settings: PortSchema="{\"entries\":[{\"content\":{\"sides\":[{\"content\":{\"connectorIds\":[\"LConn1\",\"Out1\"]},\"type\":\"ConnectorPlacement.EquallySpacedRectSide\",\"uuid\":\"bc3757cc-4537-444e-89af-7b7d8c8c1fa7\"},{\"content\":{\"connectorIds\":[\"RConn1\"],\"side\":\"RIGHT\"},\"type\":\"ConnectorPlacement.EquallySpacedRectSide\",\"uuid\":\"908bf4c4-26f6-4d8a-bcf8-68236027f5f8\"},{\"content\":{\"side\":\"TOP\"},\"type\":\"ConnectorPlacement.EquallySpacedRectSide\",\"uuid\":\"33f228db-ba47-4718-96dc-a72de309ae8c\"},{\"content\":{\"side\":\"BOTTOM\"},\"type\":\"ConnectorPlacement.EquallySpacedRectSide\",\"uuid\":\"d9b66c7e-0954-4c47-8bcc-77bf13ff573c\"}]},\"type\":\"ConnectorPlacement.EquallySpacedConnector\",\"uuid\":\"345f3578-0572-4e64-b2f3-84728129a12d\"}],\"packageUris\":[\"http://schema.mathworks.com/mf0/Connector/R2020b\"],\"version\":\"1.0\"}"
  +in : PMIOPort  Side=Right
  0 : PMIOPort  Port=2  Side=Right
  -in : PMIOPort  Port=3  Side=Right
  +out : PMIOPort  Port=4  Side=Left
  -out : PMIOPort  Port=5  Side=Left
  mDC : Outport
  wires:
  Bus Creator/1 -> mDC/1
  Vdcp/1(v) -> Bus Creator/1  "VdcpR"
  Vdcn/1(v) -> Bus Creator/2  "VdcnR"
  Sensing current1/1(i) -> Bus Creator/3  "IdcpR"
  Sensing current2/1(i) -> Bus Creator/4  "IdcnR"
  connections:
  Cfnr/LConn1 -- Cfpr/RConn1 -- Lfr/RConn1
  Lfpr/LConn1 -- Vdcp/LConn1 -- +in/RConn1 -- Cpr/LConn1 -- Cfpr/LConn1
  Cfnr/RConn1 -- Vdcn/RConn1 -- -in/RConn1 -- Cnr/RConn1 -- Lfnr/LConn1
  Sensing current1/RConn1 -- Lfpr/RConn1
  +out/RConn1 -- Sensing current1/LConn1
  Sensing current2/RConn1 -- Lfnr/RConn1
  -out/RConn1 -- Sensing current2/LConn1
  Lfr/LConn1 -- 0/RConn1 -- Vdcn/LConn1 -- Vdcp/RConn1 -- Electrical Reference/LConn1 -- Cpr/RConn1 -- Cnr/LConn1

== system VoltageSourceConverterHVDCTrans/Receiving end vi1 ==
  Current and Voltage Sensor (Three-Phase) : ee_lib/Sensors & Transducers/Current and Voltage Sensor (Three-Phase)  vMeasurementType=ee.enum.vmeasurement.lg  outputUnit=ee.enum.unit.pu  SRated=300 MW  VRated=150 kV  I_specify=off  I_priority=None  I=[0, 0, 0] A  I_nominal_specify=off  I_nominal_value=1  I_nominal_unit=A  V_specify=off  V_priority=None  V=[0, 0, 0] V  V_nominal_specify=off  V_nominal_value=1  V_nominal_unit=V
      settings: InternalSimscapePortConfiguration="{\"Bottom\":[],\"Left\":[{\"id\":\"N1\",\"label\":\"~1\",\"type\":\"foundation.electrical.three_phase\"}],\"Right\":[{\"id\":\"V_output\",\"label\":\"V\",\"type\":\"output\"},{\"id\":\"I_output\",\"label\":\"I\",\"type\":\"output\"},{\"id\":\"N2\",\"label\":\"~2\",\"type\":\"foundation.electrical.three_phase\"}],\"Top\":[]}"
  PS-Simulink Converter : nesl_utility/PS-Simulink Converter  PhysicalDomain=network_engine_domain  SubClassName=ps_output  LeftPortType=input  RightPortType=output  PseudoPeriodic=off  Frequencies=[]  VectorFormat=1-D array  Unit=1  AffineConversion=off
  PS-Simulink Converter2 : nesl_utility/PS-Simulink Converter  PhysicalDomain=network_engine_domain  SubClassName=ps_output  LeftPortType=input  RightPortType=output  PseudoPeriodic=off  Frequencies=[]  VectorFormat=1-D array  Unit=1  AffineConversion=off
  ~1 : PMIOPort  Side=Left
  ~2 : PMIOPort  Port=2  Side=Right
  v : Outport
  i : Outport  Port=2
  wires:
  PS-Simulink Converter2/1 -> v/1
  PS-Simulink Converter/1 -> i/1
  connections:
  ~2/RConn1 -- Current and Voltage Sensor (Three-Phase)/RConn3
  PS-Simulink Converter2/LConn1 -- Current and Voltage Sensor (Three-Phase)/RConn1
  Current and Voltage Sensor (Three-Phase)/RConn2 -- PS-Simulink Converter/LConn1
  Current and Voltage Sensor (Three-Phase)/LConn1 -- ~1/RConn1

== system VoltageSourceConverterHVDCTrans/Receiving end vi2 ==
  Current and Voltage Sensor (Three-Phase) : ee_lib/Sensors & Transducers/Current and Voltage Sensor (Three-Phase)  vMeasurementType=ee.enum.vmeasurement.lg  outputUnit=ee.enum.unit.pu  SRated=300 MW  VRated=345 kV  I_specify=off  I_priority=None  I=[0, 0, 0] A  I_nominal_specify=off  I_nominal_value=1  I_nominal_unit=A  V_specify=off  V_priority=None  V=[0, 0, 0] V  V_nominal_specify=off  V_nominal_value=1  V_nominal_unit=V
      settings: InternalSimscapePortConfiguration="{\"Bottom\":[],\"Left\":[{\"id\":\"N1\",\"label\":\"~1\",\"type\":\"foundation.electrical.three_phase\"}],\"Right\":[{\"id\":\"V_output\",\"label\":\"V\",\"type\":\"output\"},{\"id\":\"I_output\",\"label\":\"I\",\"type\":\"output\"},{\"id\":\"N2\",\"label\":\"~2\",\"type\":\"foundation.electrical.three_phase\"}],\"Top\":[]}"
  PS-Simulink Converter : nesl_utility/PS-Simulink Converter  PhysicalDomain=network_engine_domain  SubClassName=ps_output  LeftPortType=input  RightPortType=output  PseudoPeriodic=off  Frequencies=[]  VectorFormat=1-D array  Unit=1  AffineConversion=off
  PS-Simulink Converter2 : nesl_utility/PS-Simulink Converter  PhysicalDomain=network_engine_domain  SubClassName=ps_output  LeftPortType=input  RightPortType=output  PseudoPeriodic=off  Frequencies=[]  VectorFormat=1-D array  Unit=1  AffineConversion=off
  ~1 : PMIOPort  Side=Left
  ~2 : PMIOPort  Port=2  Side=Right
  v : Outport
  i : Outport  Port=2
  wires:
  PS-Simulink Converter/1 -> i/1
  PS-Simulink Converter2/1 -> v/1
  connections:
  Current and Voltage Sensor (Three-Phase)/LConn1 -- ~1/RConn1
  Current and Voltage Sensor (Three-Phase)/RConn2 -- PS-Simulink Converter/LConn1
  PS-Simulink Converter2/LConn1 -- Current and Voltage Sensor (Three-Phase)/RConn1
  ~2/RConn1 -- Current and Voltage Sensor (Three-Phase)/RConn3

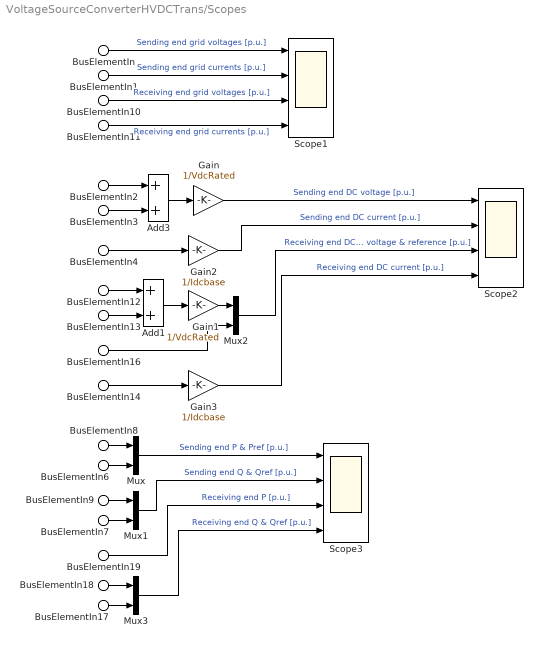
== system VoltageSourceConverterHVDCTrans/Scopes ==
  BusElementIn : Inport  PortName=mSEndAC  Element=vabcgS
  BusElementIn1 : Inport  PortName=mSEndAC  Element=iabcgS
  BusElementIn2 : Inport  Port=2  PortName=mSEndDC  Element=VdcpS
  BusElementIn3 : Inport  Port=2  PortName=mSEndDC  Element=VdcnS
  BusElementIn4 : Inport  Port=2  PortName=mSEndDC  Element=IdcpS
  BusElementIn6 : Inport  Port=3  PortName=mSEndCon  Element=Pref
  BusElementIn7 : Inport  Port=3  PortName=mSEndCon  Element=Qref
  BusElementIn8 : Inport  Port=3  PortName=mSEndCon  Element=Pmea
  BusElementIn9 : Inport  Port=3  PortName=mSEndCon  Element=Qmea
  BusElementIn10 : Inport  Port=4  PortName=mREndAC  Element=vabcgR
  BusElementIn11 : Inport  Port=4  PortName=mREndAC  Element=iabcgR
  BusElementIn12 : Inport  Port=5  PortName=mREndDC  Element=VdcpR
  BusElementIn13 : Inport  Port=5  PortName=mREndDC  Element=VdcnR
  BusElementIn14 : Inport  Port=5  PortName=mREndDC  Element=IdcpR
  BusElementIn16 : Inport  Port=6  PortName=mREndCon  Element=VdcRef
  BusElementIn17 : Inport  Port=6  PortName=mREndCon  Element=Qref
  BusElementIn18 : Inport  Port=6  PortName=mREndCon  Element=Qmea
  BusElementIn19 : Inport  Port=6  PortName=mREndCon  Element=Pmea
  Add1 : Sum
  Add3 : Sum
  Gain : Gain  Gain=1/VdcRated
  Gain1 : Gain  Gain=1/VdcRated
  Gain2 : Gain  Gain=1/Idcbase
  Gain3 : Gain  Gain=1/Idcbase
  Mux{,1..3} (4 alike) : Mux  Inputs=2
  Scope1 : Scope  NumInputPorts=4
      settings: ActiveDisplayYMinimum=-1.30664737475816  ActiveDisplayYMaximum=1.295120561976961
  Scope2 : Scope  NumInputPorts=4
      settings: ActiveDisplayYMinimum=0.90558218509651123  ActiveDisplayYMaximum=1.5317957172032071
  Scope3 : Scope  NumInputPorts=4
      settings: ActiveDisplayString=4  ActiveDisplayYMinimum=-3.7479133571511833  ActiveDisplayYMaximum=0.7531278049000969  DataLoggingVariableName=ScopeData2
  wires:
  BusElementIn2/1 -> Add3/1
  BusElementIn3/1 -> Add3/2
  Add3/1 -> Gain/1
  Add1/1 -> Gain1/1
  BusElementIn12/1 -> Add1/1
  BusElementIn13/1 -> Add1/2
  BusElementIn4/1 -> Gain2/1
  BusElementIn14/1 -> Gain3/1
  Gain/1 -> Scope2/1  "Sending end DC voltage [p.u.]"
  BusElementIn/1 -> Scope1/1  "Sending end grid voltages [p.u.]"
  BusElementIn1/1 -> Scope1/2  "Sending end grid currents [p.u.]"
  BusElementIn10/1 -> Scope1/3  "Receiving end grid voltages [p.u.]"
  BusElementIn11/1 -> Scope1/4  "Receiving end grid currents [p.u.]"
  Mux/1 -> Scope3/1  "Sending end P & Pref [p.u.]"
  Mux1/1 -> Scope3/2  "Sending end Q & Qref [p.u.]"
  Gain1/1 -> Mux2/1
  BusElementIn16/1 -> Mux2/2
  BusElementIn19/1 -> Scope3/3  "Receiving end P [p.u.]"
  BusElementIn8/1 -> Mux/1
  BusElementIn6/1 -> Mux/2
  BusElementIn7/1 -> Mux1/2
  BusElementIn9/1 -> Mux1/1
  BusElementIn18/1 -> Mux3/1
  BusElementIn17/1 -> Mux3/2
  Mux3/1 -> Scope3/4  "Receiving end Q & Qref [p.u.]"
  Gain2/1 -> Scope2/2  "Sending end DC current [p.u.]"
  Mux2/1 -> Scope2/3  "Receiving end DC voltage & reference [p.u.]"
  Gain3/1 -> Scope2/4  "Receiving end DC current [p.u.]"

== system VoltageSourceConverterHVDCTrans/Sending end Converter ==
  S : Inport
  Average-value VSC : Subsystem  VariantControl=AverageValueVSC
  Switching VSC : Subsystem  VariantControl=SwitchingVSC
  + : PMIOPort  Side=Right
  0 : PMIOPort  Port=2  Side=Right
  - : PMIOPort  Port=3  Side=Right
  ~ : PMIOPort  Port=4  Side=Left
